simulink model "Inverter_3_Phase_BIPOLAR"  (R2023b)
settings: Solver=VariableStepAuto  StartTime=0.0  StopTime=.01  RelTol=1e-3
libraries: spsMosfetLib x6, spsSeriesRLCBranchLib x3, spsVoltageMeasurementLib x2, spsDCVoltageSourceLib x1, simulink x1, sps_lib x1
settings Model: Creator=Anuj  LastModifiedBy=Anuj

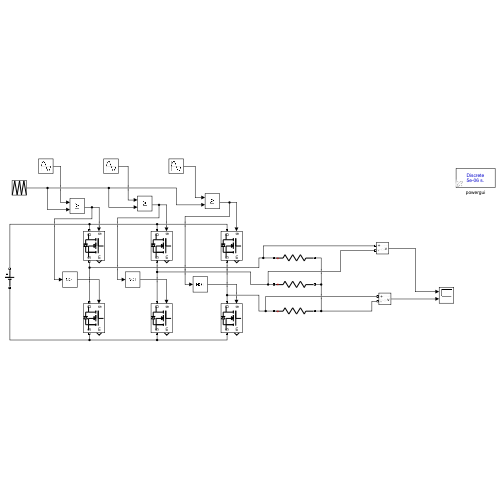
[thumbnail: Simulink's stored preview of the top-level diagram]
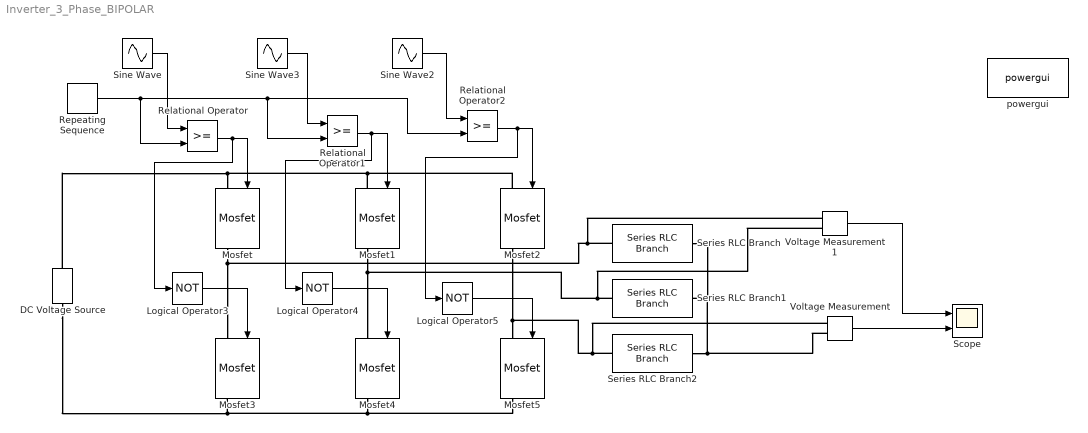
== system Inverter_3_Phase_BIPOLAR ==
  DC Voltage Source : spsDCVoltageSourceLib/DC Voltage Source  Amplitude=30  Measurements=None
  Logical Operator3 : Logic  Operator=NOT  AllPortsSameDT=off  OutDataTypeStr=boolean
  Logical Operator4 : Logic  Operator=NOT  AllPortsSameDT=off  OutDataTypeStr=boolean
  Logical Operator5 : Logic  Operator=NOT  AllPortsSameDT=off  OutDataTypeStr=boolean
  Mosfet{,1..5} (6 alike) : spsMosfetLib/Mosfet  Ron=0.1  Lon=0  Rd=0.01  Vfd=0  IC=0  Rs=1e5  Cs=inf  Measurements=on
  Relational Operator : RelationalOperator  OutDataTypeStr=boolean  RndMeth=Simplest  InputSameDT=off
  Relational Operator1 : RelationalOperator  OutDataTypeStr=boolean  RndMeth=Simplest  InputSameDT=off
  Relational Operator2 : RelationalOperator  OutDataTypeStr=boolean  RndMeth=Simplest  InputSameDT=off
  Repeating Sequence : simulink/Sources/Repeating Sequence  rep_seq_t=[0 1/40e3 1/20e3]  rep_seq_y=[-1 1 -1]
  Scope : Scope  NumInputPorts=2
  Series RLC Branch : spsSeriesRLCBranchLib/Series RLC Branch  LConnTagsString=__new0  RConnTagsString=__new0  BranchType=R  Resistance=10  Inductance=1e-3  SetiL0=off  InitialCurrent=0  Capacitance=1e-6  Setx0=off  InitialVoltage=0  Measurements=None
  Series RLC Branch1 : spsSeriesRLCBranchLib/Series RLC Branch  LConnTagsString=__new0  RConnTagsString=__new0  BranchType=R  Resistance=10  Inductance=1e-3  SetiL0=off  InitialCurrent=0  Capacitance=1e-6  Setx0=off  InitialVoltage=0  Measurements=None
  Series RLC Branch2 : spsSeriesRLCBranchLib/Series RLC Branch  LConnTagsString=__new0  RConnTagsString=__new0  BranchType=R  Resistance=10  Inductance=1e-3  SetiL0=off  InitialCurrent=0  Capacitance=1e-6  Setx0=off  InitialVoltage=0  Measurements=None
  Sine Wave : Sin  Amplitude=0.95  Frequency=50  SampleTime=0
  Sine Wave2 : Sin  Amplitude=0.95  Frequency=50  Phase=-120  SampleTime=0
  Sine Wave3 : Sin  Amplitude=0.95  Frequency=50  Phase=120  SampleTime=0
  Voltage Measurement : spsVoltageMeasurementLib/Voltage Measurement  PhasorSimulation=off  OutputType=Complex  PSBequivalent=0
  Voltage Measurement1 : spsVoltageMeasurementLib/Voltage Measurement  PhasorSimulation=off  OutputType=Complex  PSBequivalent=0
  powergui : sps_lib/powergui  Priority=1  SimulationMode=Discrete  SampleTime=1/200000  frequency=60  Iterations=50  frequencyindice=0  Pbase=100e6  ErrMax=1e-4  UnitsV=kV  UnitsW=MW  buscounter=0  FunctionMessages=off  echomessages=off  EnableUseOfTLC=off  CurrentSourceSwitches=off  DisableSnubberDevices=off  DisableRonSwitches=off  DisableVfSwitches=off  DisplayEquations=off  AutomaticDiscreteSolvers=off  SolverType=Tustin/Backward Euler (TBE)  Interpol=off  ExternalGateDelay=off  methode=off  Ts=100  x0status=blocks  SPID=on  SwTol=0  HookPort=off  NonlinearTolerance=1e-4  nMaxIteration=100  ContinueOnMaxIteration=off  RestoreLinks=warning  ResistiveCurrentMeasurement=off  Frange=[0:2:500]  Ylog=off  Xlog=on  ShowGrid=off  save=off  variable=ZData  structure=0  ZoomFFT=off  StartTime=0.0  cycles=1  DisplayStyle=1  fundamental=60  FreqAxis=off  MaxFrequency=1000  frequencyindicesteady=1  RmsSteady=1  display=off
  wires:
  Voltage Measurement/1 -> Scope/2
  Repeating Sequence/1 -> Relational Operator/2, Relational Operator2/2, Relational Operator1/2
  Sine Wave/1 -> Relational Operator/1
  Sine Wave3/1 -> Relational Operator1/1
  Sine Wave2/1 -> Relational Operator2/1
  Relational Operator/1 -> Logical Operator3/1, Mosfet/1
  Relational Operator1/1 -> Logical Operator4/1, Mosfet1/1
  Relational Operator2/1 -> Logical Operator5/1, Mosfet2/1
  Logical Operator3/1 -> Mosfet3/1
  Logical Operator4/1 -> Mosfet4/1
  Logical Operator5/1 -> Mosfet5/1
  Voltage Measurement1/1 -> Scope/1
  connections:
  DC Voltage Source/RConn1 -- Mosfet2/LConn1 -- Mosfet1/LConn1 -- Mosfet/LConn1
  DC Voltage Source/LConn1 -- Mosfet5/RConn1 -- Mosfet4/RConn1 -- Mosfet3/RConn1
  Mosfet2/RConn1 -- Voltage Measurement/LConn1 -- Series RLC Branch2/LConn1 -- Mosfet5/LConn1
  Mosfet1/RConn1 -- Voltage Measurement1/LConn2 -- Series RLC Branch1/LConn1 -- Mosfet4/LConn1
  Mosfet/RConn1 -- Voltage Measurement1/LConn1 -- Series RLC Branch/LConn1 -- Mosfet3/LConn1
  Series RLC Branch/RConn1 -- Voltage Measurement/LConn2 -- Series RLC Branch2/RConn1 -- Series RLC Branch1/RConn1
